simulink model "three_phase_inverter_v1"  (R2024a)
settings: Solver=VariableStepAuto  StartTime=0.0  StopTime=1  RelTol=1e-3
libraries: spsMosfetLib x6, spsCurrentMeasurementLib x3, spsSeriesRLCBranchLib x3, spsVoltageMeasurementLib x3, spsDCVoltageSourceLib x1, spsGroundLib x1, sps_lib x1
settings Model: Creator=Abboju Nikhil  LastModifiedBy=Abboju Nikhil

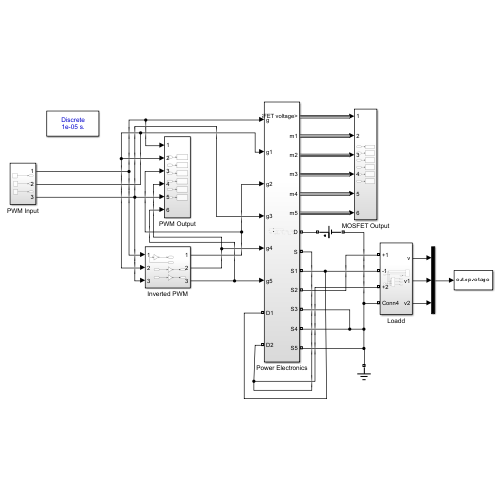
[thumbnail: Simulink's stored preview of the top-level diagram]
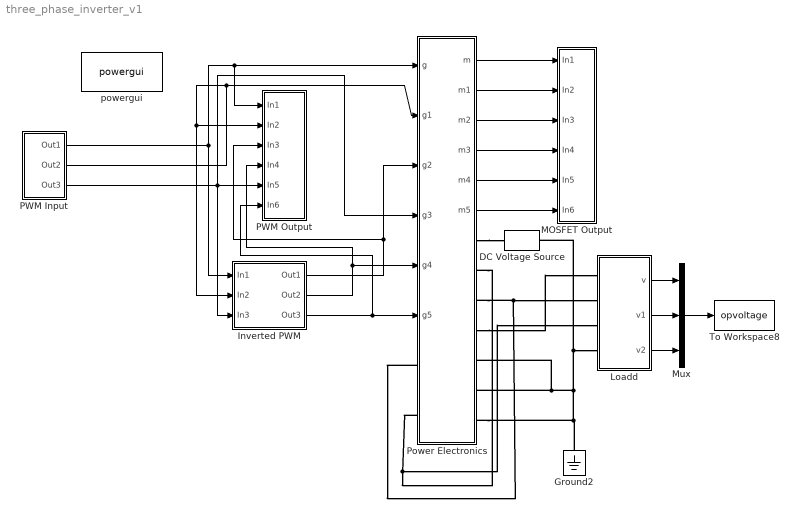
== system three_phase_inverter_v1 ==
  DC Voltage Source : spsDCVoltageSourceLib/DC Voltage Source  Amplitude=24  Measurements=None
  Ground2 : spsGroundLib/Ground  LConnTagsString=a
  Inverted PWM : Subsystem
  Loadd : Subsystem
  MOSFET Output : Subsystem
  Mux : Mux  Inputs=3
  PWM Input : Subsystem
  PWM Output : Subsystem
  Power Electronics : Subsystem
  To Workspace8 : ToWorkspace  VariableName=opvoltage  SaveFormat=Structure With Time  SampleTime=-1
  powergui : sps_lib/powergui  Priority=1  SimulationMode=Discrete  SampleTime=1E-5  frequency=60  Iterations=50  frequencyindice=0  Pbase=100e6  ErrMax=1e-4  UnitsV=kV  UnitsW=MW  buscounter=0  FunctionMessages=off  echomessages=off  EnableUseOfTLC=off  CurrentSourceSwitches=off  DisableSnubberDevices=off  DisableRonSwitches=off  DisableVfSwitches=off  DisplayEquations=off  AutomaticDiscreteSolvers=off  SolverType=Tustin/Backward Euler (TBE)  Interpol=off  ExternalGateDelay=off  methode=off  Ts=100  x0status=blocks  SPID=on  SwTol=0  HookPort=off  NonlinearTolerance=1e-4  nMaxIteration=100  ContinueOnMaxIteration=off  RestoreLinks=warning  ResistiveCurrentMeasurement=off  Frange=[0:2:500]  Ylog=off  Xlog=on  ShowGrid=off  save=off  variable=ZData  structure=0  ZoomFFT=off  StartTime=0.0  cycles=1  DisplayStyle=1  fundamental=60  FreqAxis=off  MaxFrequency=1000  frequencyindicesteady=1  RmsSteady=1  display=off
  wires:
  Inverted PWM/2(Out2) -> PWM Output/4(In4), Power Electronics/5(g4)
  PWM Input/1(Out1) -> Power Electronics/1(g), PWM Output/1(In1), Inverted PWM/1(In1)
  Inverted PWM/3(Out3) -> PWM Output/6(In6), Power Electronics/6(g5)
  PWM Input/2(Out2) -> PWM Output/2(In2), Inverted PWM/2(In2), Power Electronics/2(g1)
  PWM Input/3(Out3) -> Power Electronics/4(g3), Inverted PWM/3(In3), PWM Output/5(In5)
  Inverted PWM/1(Out1) -> Power Electronics/3(g2), PWM Output/3(In3)
  Mux/1 -> To Workspace8/1
  Power Electronics/1(m) -> MOSFET Output/1(In1)
  Power Electronics/2(m1) -> MOSFET Output/2(In2)
  Power Electronics/3(m2) -> MOSFET Output/3(In3)
  Power Electronics/4(m3) -> MOSFET Output/4(In4)
  Power Electronics/5(m4) -> MOSFET Output/5(In5)
  Power Electronics/6(m5) -> MOSFET Output/6(In6)
  Loadd/1(v) -> Mux/1
  Loadd/2(v1) -> Mux/2
  Loadd/3(v2) -> Mux/3
  connections:
  Power Electronics/RConn7 -- Ground2/LConn1 -- DC Voltage Source/LConn1 -- Loadd/LConn4 -- Power Electronics/RConn5 -- Power Electronics/RConn6
  Power Electronics/RConn1 -- DC Voltage Source/RConn1
  Power Electronics/RConn2 -- Power Electronics/LConn2 -- Loadd/LConn3
  Power Electronics/RConn3 -- Power Electronics/LConn1 -- Loadd/LConn2
  Power Electronics/RConn4 -- Loadd/LConn1

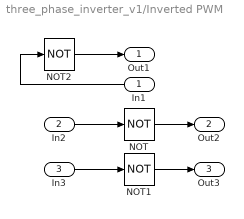
== system three_phase_inverter_v1/Inverted PWM ==
  In1 : Inport
  In2 : Inport  Port=2
  In3 : Inport  Port=3
  NOT : Logic  Operator=NOT  IconShape=distinctive  AllPortsSameDT=off  OutDataTypeStr=boolean
  NOT1 : Logic  Operator=NOT  IconShape=distinctive  AllPortsSameDT=off  OutDataTypeStr=boolean
  NOT2 : Logic  Operator=NOT  IconShape=distinctive  AllPortsSameDT=off  OutDataTypeStr=boolean
  Out1 : Outport
  Out2 : Outport  Port=2
  Out3 : Outport  Port=3
  wires:
  NOT1/1 -> Out3/1
  NOT/1 -> Out2/1
  NOT2/1 -> Out1/1
  In3/1 -> NOT1/1
  In2/1 -> NOT/1
  In1/1 -> NOT2/1

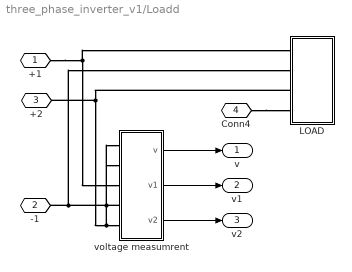
== system three_phase_inverter_v1/Loadd ==
  LOAD : Subsystem
  voltage measumrent : Subsystem
  +1 : PMIOPort  Side=Left
  -1 : PMIOPort  Port=2  Side=Left
  +2 : PMIOPort  Port=3  Side=Left
  Conn4 : PMIOPort  Port=4  Side=Left
  v : Outport
  v1 : Outport  Port=2
  v2 : Outport  Port=3
  wires:
  voltage measumrent/3(v2) -> v2/1
  voltage measumrent/2(v1) -> v1/1
  voltage measumrent/1(v) -> v/1
  connections:
  Conn4/RConn1 -- LOAD/LConn4
  +1/RConn1 -- voltage measumrent/LConn3 -- LOAD/LConn1
  voltage measumrent/LConn4 -- -1/RConn1 -- LOAD/LConn2 -- voltage measumrent/LConn2
  LOAD/LConn3 -- voltage measumrent/LConn5 -- voltage measumrent/LConn1 -- +2/RConn1

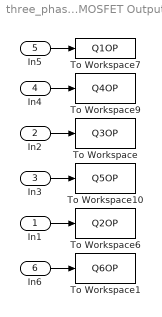
== system three_phase_inverter_v1/MOSFET Output ==
  In1 : Inport
  In2 : Inport  Port=2
  In3 : Inport  Port=3
  In4 : Inport  Port=4
  In5 : Inport  Port=5
  In6 : Inport  Port=6
  To Workspace : ToWorkspace  VariableName=Q3OP  SaveFormat=Timeseries  SampleTime=-1
  To Workspace1 : ToWorkspace  VariableName=Q6OP  SaveFormat=Timeseries  SampleTime=-1
  To Workspace10 : ToWorkspace  VariableName=Q5OP  SaveFormat=Timeseries  SampleTime=-1
  To Workspace6 : ToWorkspace  VariableName=Q2OP  SaveFormat=Timeseries  SampleTime=-1
  To Workspace7 : ToWorkspace  VariableName=Q1OP  SaveFormat=Timeseries  SampleTime=-1
  To Workspace9 : ToWorkspace  VariableName=Q4OP  SaveFormat=Timeseries  SampleTime=-1
  wires:
  In6/1 -> To Workspace1/1
  In1/1 -> To Workspace6/1
  In3/1 -> To Workspace10/1
  In2/1 -> To Workspace/1
  In4/1 -> To Workspace9/1
  In5/1 -> To Workspace7/1

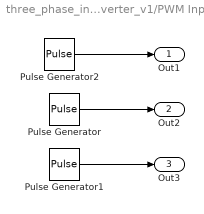
== system three_phase_inverter_v1/PWM Input ==
  Pulse Generator : DiscretePulseGenerator  PulseType=Time based  Period=0.02  PulseWidth=50
  Pulse Generator1 : DiscretePulseGenerator  PulseType=Time based  Period=0.02  PulseWidth=50  PhaseDelay=0.0066
  Pulse Generator2 : DiscretePulseGenerator  PulseType=Time based  Period=0.02  PulseWidth=50  PhaseDelay=0.0133
  Out1 : Outport
  Out2 : Outport  Port=2
  Out3 : Outport  Port=3
  wires:
  Pulse Generator1/1 -> Out3/1
  Pulse Generator/1 -> Out2/1
  Pulse Generator2/1 -> Out1/1

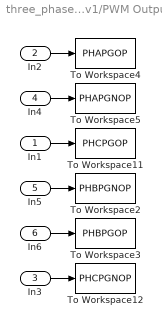
== system three_phase_inverter_v1/PWM Output ==
  In1 : Inport
  In2 : Inport  Port=2
  In3 : Inport  Port=3
  In4 : Inport  Port=4
  In5 : Inport  Port=5
  In6 : Inport  Port=6
  To Workspace11 : ToWorkspace  VariableName=PHCPGOP  SaveFormat=Structure With Time  SampleTime=-1
  To Workspace12 : ToWorkspace  VariableName=PHCPGNOP  SaveFormat=Structure With Time  SampleTime=-1
  To Workspace2 : ToWorkspace  VariableName=PHBPGNOP  SaveFormat=Structure With Time  SampleTime=-1
  To Workspace3 : ToWorkspace  VariableName=PHBPGOP  SaveFormat=Structure With Time  SampleTime=-1
  To Workspace4 : ToWorkspace  VariableName=PHAPGOP  SaveFormat=Structure With Time  SampleTime=-1
  To Workspace5 : ToWorkspace  VariableName=PHAPGNOP  SaveFormat=Structure With Time  SampleTime=-1
  wires:
  In3/1 -> To Workspace12/1
  In5/1 -> To Workspace2/1
  In1/1 -> To Workspace11/1
  In4/1 -> To Workspace5/1
  In2/1 -> To Workspace4/1
  In6/1 -> To Workspace3/1

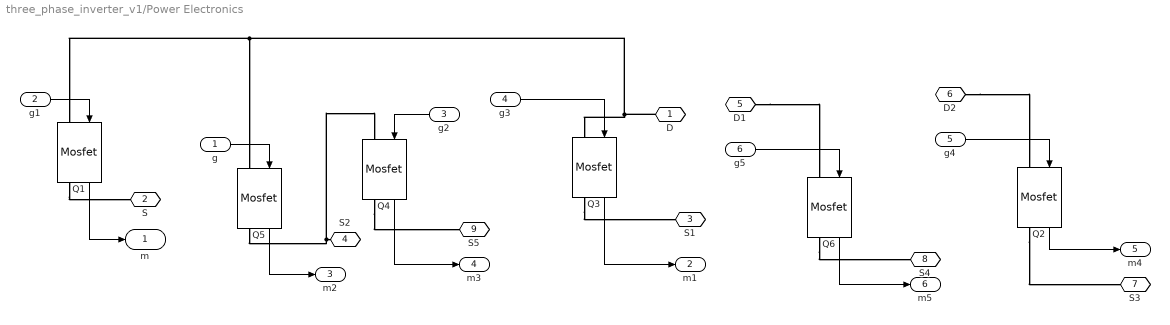
== system three_phase_inverter_v1/Power Electronics ==
  g : Inport
  g1 : Inport  Port=2
  g2 : Inport  Port=3
  g3 : Inport  Port=4
  g4 : Inport  Port=5
  g5 : Inport  Port=6
  Q{1..6} (6 alike) : spsMosfetLib/Mosfet  Ron=0.1  Lon=0  Rd=0.01  Vfd=0.8  IC=0  Rs=1e5  Cs=inf  Measurements=on
  D : PMIOPort  Side=Right
  S : PMIOPort  Port=2  Side=Right
  S1 : PMIOPort  Port=3  Side=Right
  S2 : PMIOPort  Port=4  Side=Right
  D1 : PMIOPort  Port=5  Side=Left
  D2 : PMIOPort  Port=6  Side=Left
  S3 : PMIOPort  Port=7  Side=Right
  S4 : PMIOPort  Port=8  Side=Right
  S5 : PMIOPort  Port=9  Side=Right
  m : Outport
  m1 : Outport  Port=2
  m2 : Outport  Port=3
  m3 : Outport  Port=4
  m4 : Outport  Port=5
  m5 : Outport  Port=6
  wires:
  Q6/1 -> m5/1
  g5/1 -> Q6/1
  g3/1 -> Q3/1
  Q2/1 -> m4/1
  g4/1 -> Q2/1
  g1/1 -> Q1/1
  g2/1 -> Q4/1
  g/1 -> Q5/1
  Q3/1 -> m1/1
  Q5/1 -> m2/1
  Q1/1 -> m/1
  Q4/1 -> m3/1
  connections:
  D/RConn1 -- Q3/LConn1 -- Q1/LConn1 -- Q5/LConn1
  D1/RConn1 -- Q6/LConn1
  Q6/RConn1 -- S4/RConn1
  D2/RConn1 -- Q2/LConn1
  Q2/RConn1 -- S3/RConn1
  Q5/RConn1 -- Q4/LConn1 -- S2/RConn1
  Q3/RConn1 -- S1/RConn1
  Q1/RConn1 -- S/RConn1
  Q4/RConn1 -- S5/RConn1

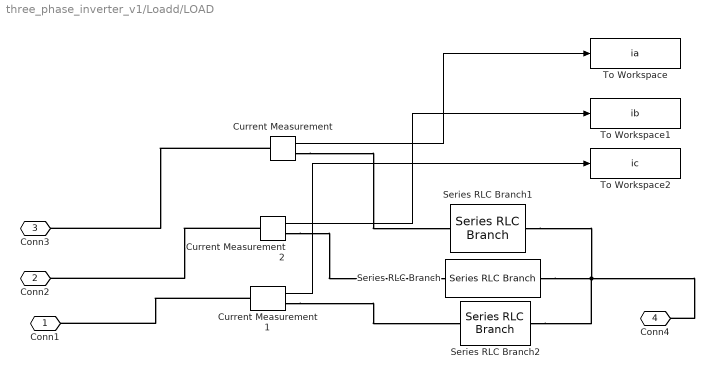
== system three_phase_inverter_v1/Loadd/LOAD ==
  Current Measurement : spsCurrentMeasurementLib/Current Measurement  PhasorSimulation=off  OutputType=Complex  PSBequivalent=0
  Current Measurement1 : spsCurrentMeasurementLib/Current Measurement  PhasorSimulation=off  OutputType=Complex  PSBequivalent=0
  Current Measurement2 : spsCurrentMeasurementLib/Current Measurement  PhasorSimulation=off  OutputType=Complex  PSBequivalent=0
  Series RLC Branch : spsSeriesRLCBranchLib/Series RLC Branch  LConnTagsString=__new0  RConnTagsString=__new0  BranchType=R  Resistance=10000  Inductance=1e-3  SetiL0=off  InitialCurrent=0  Capacitance=1e-6  Setx0=off  InitialVoltage=0  Measurements=None
  Series RLC Branch1 : spsSeriesRLCBranchLib/Series RLC Branch  LConnTagsString=__new0  RConnTagsString=__new0  BranchType=R  Resistance=10000  Inductance=1e-3  SetiL0=off  InitialCurrent=0  Capacitance=1e-6  Setx0=off  InitialVoltage=0  Measurements=None
  Series RLC Branch2 : spsSeriesRLCBranchLib/Series RLC Branch  LConnTagsString=__new0  RConnTagsString=__new0  BranchType=R  Resistance=10000  Inductance=1e-3  SetiL0=off  InitialCurrent=0  Capacitance=1e-6  Setx0=off  InitialVoltage=0  Measurements=None
  To Workspace : ToWorkspace  VariableName=ia  SaveFormat=Timeseries  SampleTime=-1
  To Workspace1 : ToWorkspace  VariableName=ib  SaveFormat=Timeseries  SampleTime=-1
  To Workspace2 : ToWorkspace  VariableName=ic  SaveFormat=Timeseries  SampleTime=-1
  Conn1 : PMIOPort  Side=Left
  Conn2 : PMIOPort  Port=2  Side=Left
  Conn3 : PMIOPort  Port=3  Side=Left
  Conn4 : PMIOPort  Port=4  Side=Left
  wires:
  Current Measurement/1 -> To Workspace/1
  Current Measurement2/1 -> To Workspace1/1
  Current Measurement1/1 -> To Workspace2/1
  connections:
  Series RLC Branch/RConn1 -- Conn4/RConn1 -- Series RLC Branch1/RConn1 -- Series RLC Branch2/RConn1
  Current Measurement1/LConn1 -- Conn1/RConn1
  Current Measurement/LConn1 -- Conn3/RConn1
  Current Measurement/RConn1 -- Series RLC Branch1/LConn1
  Current Measurement2/LConn1 -- Conn2/RConn1
  Current Measurement2/RConn1 -- Series RLC Branch/LConn1
  Current Measurement1/RConn1 -- Series RLC Branch2/LConn1

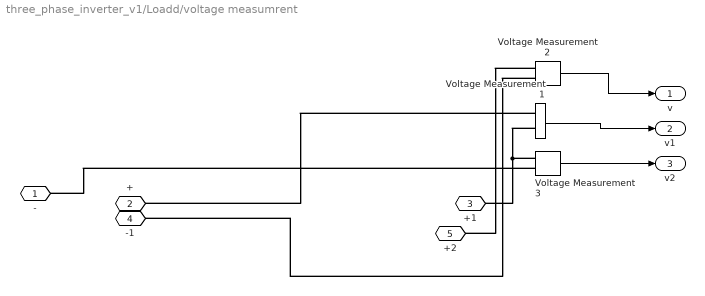
== system three_phase_inverter_v1/Loadd/voltage measumrent ==
  Voltage Measurement1 : spsVoltageMeasurementLib/Voltage Measurement  PhasorSimulation=off  OutputType=Complex  PSBequivalent=0
  Voltage Measurement2 : spsVoltageMeasurementLib/Voltage Measurement  PhasorSimulation=off  OutputType=Complex  PSBequivalent=0
  Voltage Measurement3 : spsVoltageMeasurementLib/Voltage Measurement  PhasorSimulation=off  OutputType=Complex  PSBequivalent=0
  - : PMIOPort  Side=Left
  + : PMIOPort  Port=2  Side=Left
  +1 : PMIOPort  Port=3  Side=Left
  -1 : PMIOPort  Port=4  Side=Left
  +2 : PMIOPort  Port=5  Side=Left
  v : Outport
  v1 : Outport  Port=2
  v2 : Outport  Port=3
  wires:
  Voltage Measurement1/1 -> v1/1
  Voltage Measurement2/1 -> v/1
  Voltage Measurement3/1 -> v2/1
  connections:
  Voltage Measurement3/LConn2 -- -/RConn1
  Voltage Measurement1/LConn1 -- +/RConn1
  Voltage Measurement1/LConn2 -- +1/RConn1 -- Voltage Measurement3/LConn1
  Voltage Measurement2/LConn1 -- +2/RConn1
  Voltage Measurement2/LConn2 -- -1/RConn1
